simulink model "PV_simulation"  (R2024b)
settings: Solver=VariableStepAuto  StartTime=0.0  StopTime=6  RelTol=1e-3
undefined symbols (not defined in the file or in its folder): DiscIntNeverNeededParam, dspblkCoreblockFVToolHelper, gcbh, Ion, Lithium
libraries: spsSeriesRLCBranchLib x3, simulink x2, spsBatteryLib x1, spsDiodeLib x1, eePwmGenerator x1, spsMosfetLib x1, spsPVArrayLib x1, sps_lib x1
settings Model: Creator=nikul  LastModifiedBy=nikul

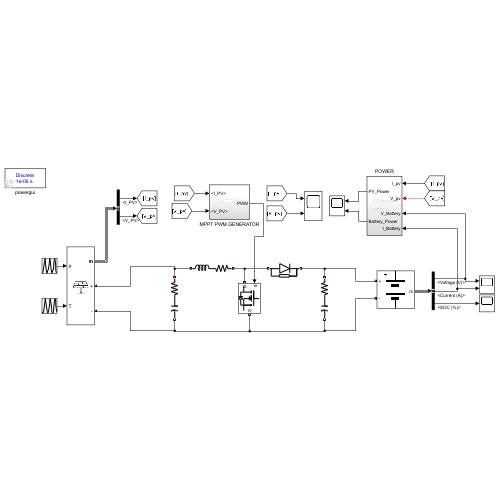
[thumbnail: Simulink's stored preview of the top-level diagram]
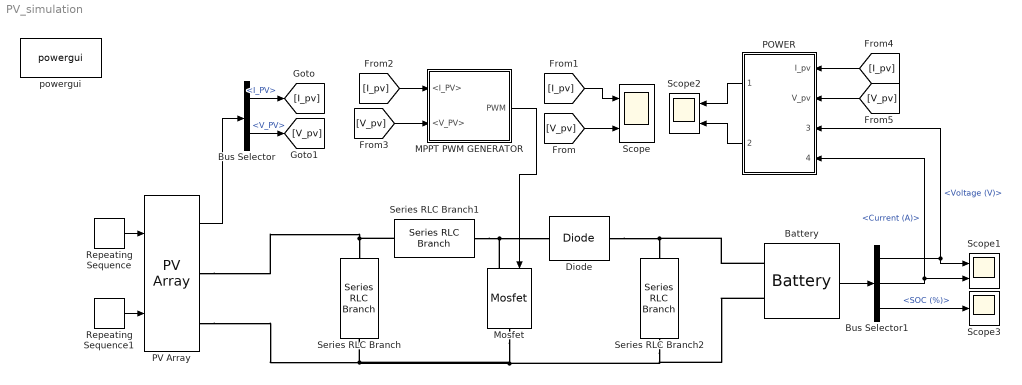
== system PV_simulation ==
  Battery : spsBatteryLib/Battery  BatType=Lithium-Ion  NomV=48  NomQ=20  SOC=50  Batt_Tr=1  PresetModel=on  MaxQ=20  MinV=36  FullV=55.8714  Dis_rate=8.6957  R=0.024  Normal_OP=18.087  expZone="[51.8585     0.982609]"
  Bus Selector : BusSelector  OutputSignals=I_PV,V_PV
  Bus Selector1 : BusSelector  OutputSignals=Voltage (V),Current (A),SOC (%)
  Diode : spsDiodeLib/Diode  Ron=0.001  Lon=0  Vf=0.8  IC=0  UseSnubber=0  Rs=500  Cs=250e-9  Measurements=off
  MPPT PWM GENERATOR : Subsystem
  Mosfet : spsMosfetLib/Mosfet  Ron=0.1  Lon=0  Rd=0.01  Vfd=0  IC=0  Rs=1e5  Cs=inf  Measurements=off
  POWER : Subsystem
  PV Array : spsPVArrayLib/PV Array  Npar=1  Nser=1  PlotType=array @ 1000 W/m2 & specified temperatures  S_vec="[ 1000  500  100 ]"  Temp_C_vec="[ 45 25  ]"  ModuleName=Trina Solar TSM-250PA05.18  PlotWhenSelected=off  Pm=249.86  Ncell=60  Voc=37.6  Isc=8.55  Vm=31  Im=8.06  beta_Voc_pc=-0.35  alpha_Isc_pc=0.06  beta_Voc=-0.1316  alpha_Isc=0.00513  IL=8.5795  I0=2.0381e-10  nI=0.99766  Rsh=301.8149  Rs=0.247  RobustModel=off  RobustCellTemperature=313.3991  BAL=on  Tc=1e-6  Tfilter=5e-5
  Repeating Sequence : simulink/Sources/Repeating Sequence  rep_seq_t=[0 0.5 1 1.5 2 2.5 3 3.5 4 4.5 5 5.5 6]  rep_seq_y=[0 20 200 200 400 700 900 1000 850 500 200 20 0]
  Repeating Sequence1 : simulink/Sources/Repeating Sequence  rep_seq_t=[0 0.5 1 1.5 2 2.5 3 3.5 4 4.5 5 5.5 6]  rep_seq_y=[26 25 24 25 29 35 42 48 50 45 38 32 28]
  Scope : Scope  NumInputPorts=2
  Scope1 : Scope  NumInputPorts=2
  Scope2 : Scope  NumInputPorts=2
  Scope3 : Scope
  Series RLC Branch : spsSeriesRLCBranchLib/Series RLC Branch  LConnTagsString=__new0  RConnTagsString=__new0  BranchType=RC  Resistance=0.4  Inductance=1e-3  SetiL0=off  InitialCurrent=0  Capacitance=300e-6  Setx0=off  InitialVoltage=0  Measurements=None
  Series RLC Branch1 : spsSeriesRLCBranchLib/Series RLC Branch  LConnTagsString=__new0  RConnTagsString=__new0  BranchType=RL  Resistance=0.02  Inductance=450e-6  SetiL0=off  InitialCurrent=0  Capacitance=100e-6  Setx0=off  InitialVoltage=0  Measurements=None
  Series RLC Branch2 : spsSeriesRLCBranchLib/Series RLC Branch  LConnTagsString=__new0  RConnTagsString=__new0  BranchType=RC  Resistance=0.05  Inductance=1e-3  SetiL0=off  InitialCurrent=0  Capacitance=1500e-6  Setx0=on  InitialVoltage=46  Measurements=None
  powergui : sps_lib/powergui  Priority=1  SimulationMode=Discrete  SampleTime=1e-6  frequency=60  Iterations=50  frequencyindice=0  Pbase=100e6  ErrMax=1e-4  UnitsV=kV  UnitsW=MW  buscounter=0  FunctionMessages=off  echomessages=off  EnableUseOfTLC=off  CurrentSourceSwitches=off  DisableSnubberDevices=off  DisableRonSwitches=off  DisableVfSwitches=off  DisplayEquations=off  AutomaticDiscreteSolvers=off  SolverType=Tustin/Backward Euler (TBE)  Interpol=off  ExternalGateDelay=off  methode=off  Ts=100  x0status=blocks  SPID=on  SwTol=0  HookPort=off  NonlinearTolerance=1e-4  nMaxIteration=100  ContinueOnMaxIteration=off  RestoreLinks=warning  ResistiveCurrentMeasurement=off  Frange=[0:2:500]  Ylog=off  Xlog=on  ShowGrid=off  save=off  variable=ZData  structure=0  ZoomFFT=off  StartTime=0.0  cycles=1  DisplayStyle=1  fundamental=60  FreqAxis=off  MaxFrequency=1000  frequencyindicesteady=1  RmsSteady=1  display=off
  wires:
  PV Array/1 -> Bus Selector/1
  Battery/1 -> Bus Selector1/1
  Bus Selector1/1 -> Scope1/1, POWER/3(V_Battery)  "<Voltage (V)>"
  Bus Selector1/2 -> POWER/4(I_Battery), Scope1/2  "<Current (A)>"
  Bus Selector1/3 -> Scope3/1  "<SOC (%)>"
  Bus Selector/1 -> [I_pv]  "<I_PV>"
  Bus Selector/2 -> [V_pv]  "<V_PV>"
  [I_pv] -> Scope/1
  [V_pv] -> Scope/2
  [I_pv] -> MPPT PWM GENERATOR/1(<I_PV>)
  [V_pv] -> MPPT PWM GENERATOR/2(<V_PV>)
  [I_pv] -> POWER/1(I_pv)
  [V_pv] -> POWER/2(V_pv)
  POWER/1(PV_Power) -> Scope2/1
  POWER/2(Battery_Power) -> Scope2/2
  MPPT PWM GENERATOR/1(PWM) -> Mosfet/1
  Repeating Sequence/1 -> PV Array/1
  Repeating Sequence1/1 -> PV Array/2
  connections:
  PV Array/RConn1 -- Series RLC Branch/LConn1 -- Series RLC Branch1/RConn1
  Diode/RConn1 -- Battery/LConn1 -- Series RLC Branch2/LConn1
  PV Array/RConn2 -- Series RLC Branch/RConn1 -- Battery/LConn2 -- Series RLC Branch2/RConn1 -- Mosfet/RConn1
  Mosfet/LConn1 -- Series RLC Branch1/LConn1 -- Diode/LConn1

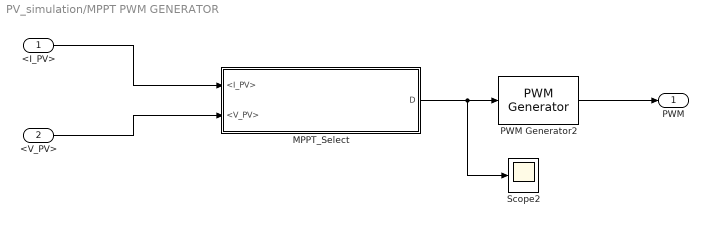
== system PV_simulation/MPPT PWM GENERATOR ==
  <I_PV> : Inport
  <V_PV> : Inport  Port=2
  MPPT_Select : Subsystem  Variant=on
  PWM Generator2 : eePwmGenerator/PWM Generator  CarrCount=Up  Tper=1e-4  Tdelay=0  Ts=1e-6
  Scope2 : Scope
  PWM : Outport
  wires:
  <I_PV>/1 -> MPPT_Select/1(<I_PV>)
  <V_PV>/1 -> MPPT_Select/2(<V_PV>)
  MPPT_Select/1(D) -> Scope2/1, PWM Generator2/1
  PWM Generator2/1 -> PWM/1

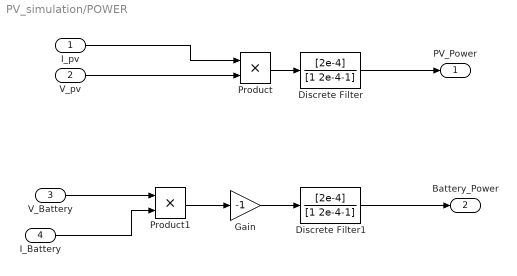
== system PV_simulation/POWER ==
  I_pv : Inport
  V_pv : Inport  Port=2
  V_Battery : Inport  Port=3
  I_Battery : Inport  Port=4
  Discrete Filter : DiscreteFilter  LoadFcn=dspblkCoreblockFVToolHelper(gcbh,'load');  Numerator=[2e-4]  Denominator=[1 2e-4-1]
      settings: CopyFcn=dspblkCoreblockFVToolHelper(gcbh,'copy');  DeleteFcn=dspblkCoreblockFVToolHelper(gcbh,'close');  ModelCloseFcn=dspblkCoreblockFVToolHelper(gcbh,'close');  PreSaveFcn=dspblkCoreblockFVToolHelper(gcbh,'presave');  PostSaveFcn=dspblkCoreblockFVToolHelper(gcbh,'postsave');  CloseFcn=dspblkCoreblockFVToolHelper(gcbh,'close');
  Discrete Filter1 : DiscreteFilter  LoadFcn=dspblkCoreblockFVToolHelper(gcbh,'load');  Numerator=[2e-4]  Denominator=[1 2e-4-1]
      settings: CopyFcn=dspblkCoreblockFVToolHelper(gcbh,'copy');  DeleteFcn=dspblkCoreblockFVToolHelper(gcbh,'close');  ModelCloseFcn=dspblkCoreblockFVToolHelper(gcbh,'close');  PreSaveFcn=dspblkCoreblockFVToolHelper(gcbh,'presave');  PostSaveFcn=dspblkCoreblockFVToolHelper(gcbh,'postsave');  CloseFcn=dspblkCoreblockFVToolHelper(gcbh,'close');
  Gain : Gain  Gain=-1
  Product : Product
  Product1 : Product
  PV_Power : Outport
  Battery_Power : Outport  Port=2
  wires:
  Discrete Filter1/1 -> Battery_Power/1
  Product/1 -> Discrete Filter/1
  Product1/1 -> Gain/1
  Gain/1 -> Discrete Filter1/1
  V_pv/1 -> Product/2
  V_Battery/1 -> Product1/1
  Discrete Filter/1 -> PV_Power/1
  I_pv/1 -> Product/1
  I_Battery/1 -> Product1/2

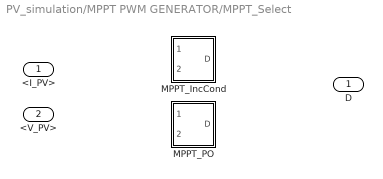
== system PV_simulation/MPPT PWM GENERATOR/MPPT_Select ==
  <I_PV> : Inport
  <V_PV> : Inport  Port=2
  MPPT_IncCond : Subsystem  VariantControl=MPPT_ALGO == 1
  MPPT_PO : Subsystem  VariantControl=MPPT_ALGO == 2
  D : Outport

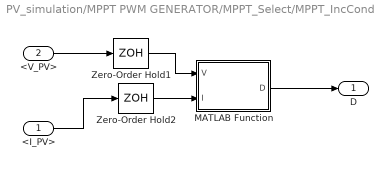
== system PV_simulation/MPPT PWM GENERATOR/MPPT_Select/MPPT_IncCond ==
  <I_PV> : Inport
  <V_PV> : Inport  Port=2
  MATLAB Function : MATLAB Function  TreatAsAtomicUnit=on
  Zero-Order Hold1 : ZeroOrderHold  SampleTime=0.02
  Zero-Order Hold2 : ZeroOrderHold  SampleTime=0.02
  D : Outport
  wires:
  <V_PV>/1 -> Zero-Order Hold1/1
  <I_PV>/1 -> Zero-Order Hold2/1
  MATLAB Function/1(D) -> D/1
  Zero-Order Hold1/1 -> MATLAB Function/1(V)
  Zero-Order Hold2/1 -> MATLAB Function/2(I)

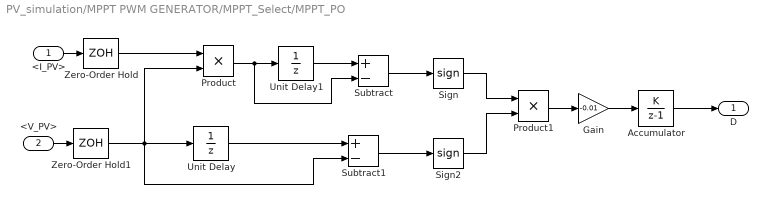
== system PV_simulation/MPPT PWM GENERATOR/MPPT_Select/MPPT_PO ==
  <I_PV> : Inport
  <V_PV> : Inport  Port=2
  Accumulator : DiscreteIntegrator  IntegratorMethod=Accumulation: Forward Euler  InitialCondition=0.5  SampleTime=-1  LimitOutput=on  UpperSaturationLimit=0.95  LowerSaturationLimit=0.05  ICPrevOutput=DiscIntNeverNeededParam  ICPrevScaledInput=DiscIntNeverNeededParam
  Gain : Gain  Gain=-0.01
  Product : Product
  Product1 : Product
  Sign : Signum
  Sign2 : Signum
  Subtract : Sum  Inputs=+-
  Subtract1 : Sum  Inputs=+-
  Unit Delay : UnitDelay  SampleTime=-1  HasFrameUpgradeWarning=on
  Unit Delay1 : UnitDelay  SampleTime=-1  HasFrameUpgradeWarning=on
  Zero-Order Hold : ZeroOrderHold  SampleTime=0.02
  Zero-Order Hold1 : ZeroOrderHold  SampleTime=0.02
  D : Outport
  wires:
  Unit Delay/1 -> Subtract1/1
  Sign2/1 -> Product1/2
  Zero-Order Hold1/1 -> Unit Delay/1, Product/2, Subtract1/2
  Zero-Order Hold/1 -> Product/1
  Sign/1 -> Product1/1
  Unit Delay1/1 -> Subtract/1
  Product/1 -> Subtract/2, Unit Delay1/1
  Subtract/1 -> Sign/1
  Subtract1/1 -> Sign2/1
  Product1/1 -> Gain/1
  Gain/1 -> Accumulator/1
  Accumulator/1 -> D/1
  <V_PV>/1 -> Zero-Order Hold1/1
  <I_PV>/1 -> Zero-Order Hold/1

== matlab function PV_simulation/MPPT PWM GENERATOR/MPPT_Select/MPPT_IncCond/MATLAB Function ==
  data: V input; D output; I input
function D = incCond(V, I)
    persistent Vp Ip Dp
    if isempty(Vp), Vp = V; Ip = I; Dp = 0.5; end

    step = 0.002;  Dmin = 0.2;  Dmax = 0.8;
    D  = Dp;
    I  = max(I, 0);                 % ignore negative current spikes

    if V > 5 && V*I > 1             % only track when there is real power
        dV = V - Vp;  dI = I - Ip;
        if abs(dV) < 0.02
            if abs(dI) < 0.01
                % hold
            elseif dI > 0
                D = Dp - step;
            else
                D = Dp + step;
            end
        else
            err = dI/dV + I/V;
            if abs(err) < 0.01*(I/V)    % relative deadband
                % hold
            elseif err > 0
                D = Dp - step;
            else
                D = Dp + step;
            end
        end
    end

    D  = min(max(D, Dmin), Dmax);
    Vp = V;  Ip = I;  Dp = D;
end
